simulink model "Inverter_3_Phase_180_Conduction"  (R2023b)
settings: Solver=VariableStepAuto  StartTime=0.0  StopTime=0.01  RelTol=1e-3
libraries: spsMosfetLib x6, spsSeriesRLCBranchLib x3, spsVoltageMeasurementLib x2, spsDCVoltageSourceLib x1, sps_lib x1
settings Model: Creator=Anuj  LastModifiedBy=Anuj

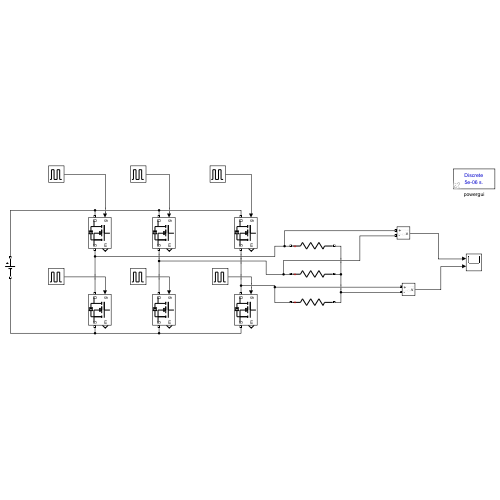
[thumbnail: Simulink's stored preview of the top-level diagram]
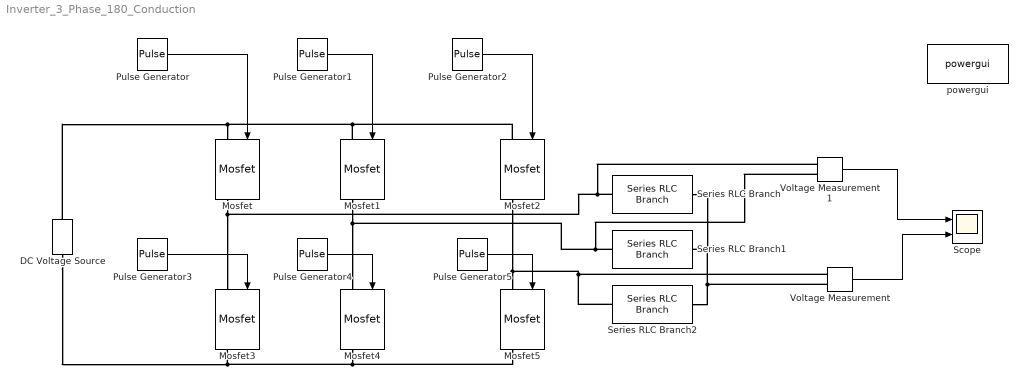
== system Inverter_3_Phase_180_Conduction ==
  DC Voltage Source : spsDCVoltageSourceLib/DC Voltage Source  Amplitude=30  Measurements=None
  Mosfet{,1..5} (6 alike) : spsMosfetLib/Mosfet  Ron=0.1  Lon=0  Rd=0.01  Vfd=0  IC=0  Rs=1e5  Cs=inf  Measurements=on
  Pulse Generator : DiscretePulseGenerator  PulseType=Time based  Period=1/20000  PulseWidth=50
  Pulse Generator1 : DiscretePulseGenerator  PulseType=Time based  Period=1/20000  PulseWidth=50  PhaseDelay=(120/360)*(1/20000)
  Pulse Generator2 : DiscretePulseGenerator  PulseType=Time based  Period=1/20000  PulseWidth=50  PhaseDelay=(240/360)*(1/20000)
  Pulse Generator3 : DiscretePulseGenerator  PulseType=Time based  Period=1/20000  PulseWidth=50  PhaseDelay=(180/360)*(1/20000)
  Pulse Generator4 : DiscretePulseGenerator  PulseType=Time based  Period=1/20000  PulseWidth=50  PhaseDelay=(300/360)*(1/20000)
  Pulse Generator5 : DiscretePulseGenerator  PulseType=Time based  Period=1/20000  PulseWidth=50  PhaseDelay=(420/360)*(1/20000)
  Scope : Scope  NumInputPorts=2
  Series RLC Branch : spsSeriesRLCBranchLib/Series RLC Branch  LConnTagsString=__new0  RConnTagsString=__new0  BranchType=R  Resistance=10  Inductance=1e-3  SetiL0=off  InitialCurrent=0  Capacitance=1e-6  Setx0=off  InitialVoltage=0  Measurements=None
  Series RLC Branch1 : spsSeriesRLCBranchLib/Series RLC Branch  LConnTagsString=__new0  RConnTagsString=__new0  BranchType=R  Resistance=10  Inductance=1e-3  SetiL0=off  InitialCurrent=0  Capacitance=1e-6  Setx0=off  InitialVoltage=0  Measurements=None
  Series RLC Branch2 : spsSeriesRLCBranchLib/Series RLC Branch  LConnTagsString=__new0  RConnTagsString=__new0  BranchType=R  Resistance=10  Inductance=1e-3  SetiL0=off  InitialCurrent=0  Capacitance=1e-6  Setx0=off  InitialVoltage=0  Measurements=None
  Voltage Measurement : spsVoltageMeasurementLib/Voltage Measurement  PhasorSimulation=off  OutputType=Complex  PSBequivalent=0
  Voltage Measurement1 : spsVoltageMeasurementLib/Voltage Measurement  PhasorSimulation=off  OutputType=Complex  PSBequivalent=0
  powergui : sps_lib/powergui  Priority=1  SimulationMode=Discrete  SampleTime=1/200000  frequency=60  Iterations=50  frequencyindice=0  Pbase=100e6  ErrMax=1e-4  UnitsV=kV  UnitsW=MW  buscounter=0  FunctionMessages=off  echomessages=off  EnableUseOfTLC=off  CurrentSourceSwitches=off  DisableSnubberDevices=off  DisableRonSwitches=off  DisableVfSwitches=off  DisplayEquations=off  AutomaticDiscreteSolvers=off  SolverType=Tustin/Backward Euler (TBE)  Interpol=off  ExternalGateDelay=off  methode=off  Ts=100  x0status=blocks  SPID=on  SwTol=0  HookPort=off  NonlinearTolerance=1e-4  nMaxIteration=100  ContinueOnMaxIteration=off  RestoreLinks=warning  ResistiveCurrentMeasurement=off  Frange=[0:2:500]  Ylog=off  Xlog=on  ShowGrid=off  save=off  variable=ZData  structure=0  ZoomFFT=off  StartTime=0.0  cycles=1  DisplayStyle=1  fundamental=60  FreqAxis=off  MaxFrequency=1000  frequencyindicesteady=1  RmsSteady=1  display=off
  wires:
  Pulse Generator/1 -> Mosfet/1
  Pulse Generator1/1 -> Mosfet1/1
  Pulse Generator2/1 -> Mosfet2/1
  Pulse Generator3/1 -> Mosfet3/1
  Pulse Generator4/1 -> Mosfet4/1
  Pulse Generator5/1 -> Mosfet5/1
  Voltage Measurement/1 -> Scope/2
  Voltage Measurement1/1 -> Scope/1
  connections:
  DC Voltage Source/RConn1 -- Mosfet2/LConn1 -- Mosfet1/LConn1 -- Mosfet/LConn1
  DC Voltage Source/LConn1 -- Mosfet5/RConn1 -- Mosfet4/RConn1 -- Mosfet3/RConn1
  Mosfet2/RConn1 -- Series RLC Branch2/LConn1 -- Voltage Measurement/LConn1 -- Mosfet5/LConn1
  Mosfet1/RConn1 -- Voltage Measurement1/LConn2 -- Series RLC Branch1/LConn1 -- Mosfet4/LConn1
  Mosfet/RConn1 -- Voltage Measurement1/LConn1 -- Series RLC Branch/LConn1 -- Mosfet3/LConn1
  Series RLC Branch/RConn1 -- Voltage Measurement/LConn2 -- Series RLC Branch2/RConn1 -- Series RLC Branch1/RConn1
